simulink model "dab_openloop_variable_step"  (R2024b)
settings: Solver=ode1be  StartTime=0.0  StopTime=T_stop  FixedStep=TFIX  MaxStep=Tsolver  RelTol=1e-05
values from neighbouring files (symbols this model uses):
  Ci = 30e-6*s_f    (= 7.5e-05)    [init.m]
  Co = 44e-6*s_f    (= 0.00011)    [init.m]
  D1_OL = 0.985714    [init.m]
  D2_OL = 1    [init.m]
  D3_OL = 0.045188    [init.m]
  ESR_Ci = 2e-3    (= 0.002)    [init.m]
  ESR_Co = 2e-3    (= 0.002)    [init.m]
  f_sw = 20e3    (= 20000)    [init.m]
  Li = 10e-6*s_f    (= 2.5e-05)    [init.m]
  Lo = 10e-6*s_f    (= 2.5e-05)    [init.m]
  Ri = 100e-3    (= 0.1)    [init.m]
  Ro = 100e-3    (= 0.1)    [init.m]
  tdead = 200e-9    (= 2e-07)    [init.m]
  TR_fn = f_sw    (= 20000)    [init.m]
  TR_Lm = 1    [init.m]
  TR_Pn = 30e3    (= 30000)    [init.m]
  TR_Rm = 1e6    (= 1000000)    [init.m]
  Vi = 800    [init.m]
  Vo = V_BAT    (= 450)    [init.m]
libraries: spsMosfetLib x8, spsSeriesRLCBranchLib x4, spsControlledVoltageSourceLib x2, spsCurrentMeasurementLib x2, spsGroundLib x2, spsVoltageMeasurementLib x2, spsLinearTransformerLib x1, sps_lib x1
settings Model: Creator=amina  LastModifiedBy=amina
settings SolverCC: MaxConsecutiveMinStep=100
settings DataIOCC: SaveOutput=off  SignalLogging=off  DSMLogging=off  SaveTime=off  ReturnWorkspaceOutputsName=out_analytic

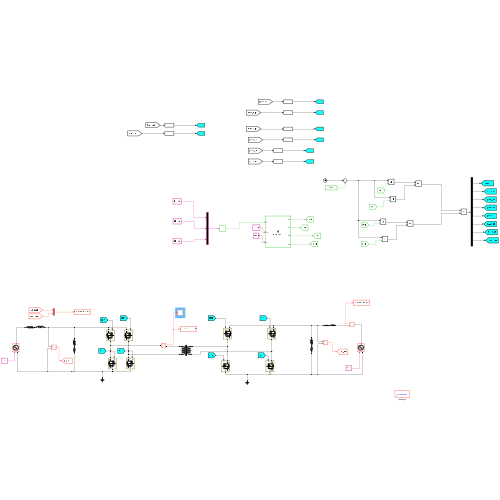
[thumbnail: Simulink's stored preview of the top-level diagram]
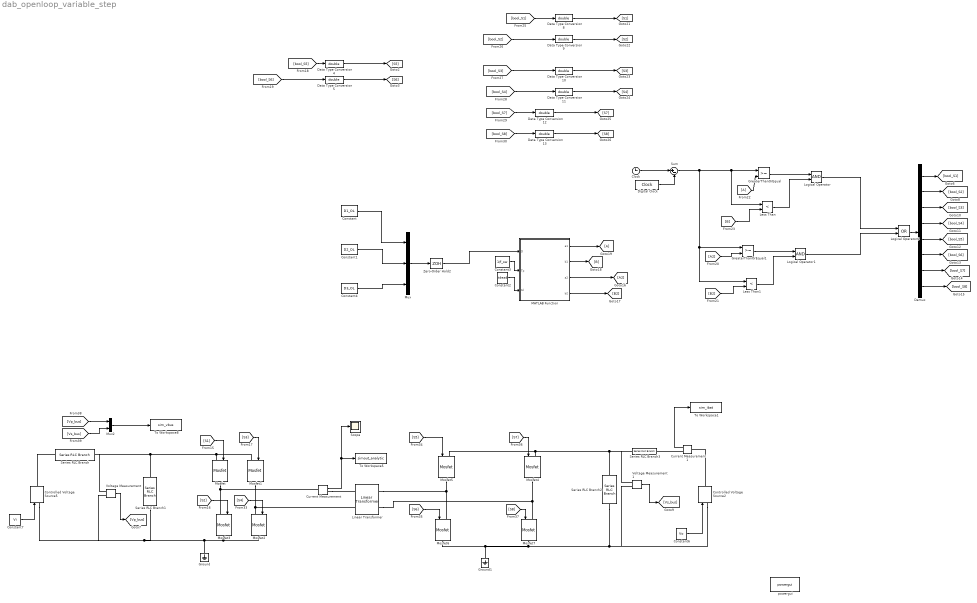
== system dab_openloop_variable_step ==
  Clock : Clock
  Constant : Constant  Value=D1_OL
  Constant1 : Constant  Value=D2_OL
  Constant2 : Constant  Value=tdead
  Constant3 : Constant  Value=1/f_sw
  Constant4 : Constant  Value=D3_OL
  Constant6 : Constant  Value=Vo
  Constant7 : Constant  Value=Vi
  Controlled Voltage Source2 : spsControlledVoltageSourceLib/Controlled Voltage Source  Initialize=on  Source_Type=DC  Amplitude=Vo  Phase=0  Frequency=0  Measurements=None
  Controlled Voltage Source5 : spsControlledVoltageSourceLib/Controlled Voltage Source  Initialize=on  Source_Type=DC  Amplitude=Vi  Phase=0  Frequency=0  Measurements=None
  Current Measurement : spsCurrentMeasurementLib/Current Measurement  PhasorSimulation=off  OutputType=Complex  PSBequivalent=0
  Current Measurement1 : spsCurrentMeasurementLib/Current Measurement  PhasorSimulation=off  OutputType=Complex  PSBequivalent=0
  Data Type Conversion{4..5,8..13} (8 alike) : DataTypeConversion  OutDataTypeStr=double  SaturateOnIntegerOverflow=off  RndMeth=Floor
  Demux : Demux  Outputs=8
  Digital Clock : DigitalClock  SampleTime=1/f_sw
  From22 : From
  Goto19 : Goto
  GreaterThanOrEqual : RelationalOperator  OutDataTypeStr=boolean  RndMeth=Simplest  InputSameDT=off
  GreaterThanOrEqual1 : RelationalOperator  OutDataTypeStr=boolean  RndMeth=Simplest  InputSameDT=off
  Ground : spsGroundLib/Ground  LConnTagsString=a
  Ground1 : spsGroundLib/Ground  LConnTagsString=a
  Less Than : RelationalOperator  Operator=<  OutDataTypeStr=boolean  RndMeth=Simplest  InputSameDT=off
  Less Than1 : RelationalOperator  Operator=<  OutDataTypeStr=boolean  RndMeth=Simplest  InputSameDT=off
  Linear Transformer : spsLinearTransformerLib/Linear Transformer  UNITS=SI  NominalPower=[TR_Pn TR_fn]  winding1=TR_W1  winding2=TR_W2  ThreeWindings=off  winding3=[3.15e+05 0.7938 0.084225]  RmLm=[TR_Rm TR_Lm]  Measurements=None  DataType=on
  Logical Operator : Logic  AllPortsSameDT=off  OutDataTypeStr=boolean
  Logical Operator1 : Logic  AllPortsSameDT=off  OutDataTypeStr=boolean
  Logical Operator6 : Logic  Operator=OR  AllPortsSameDT=off  OutDataTypeStr=boolean
  MATLAB Function : MATLAB Function  TreatAsAtomicUnit=on
  Mosfet{,1..7} (8 alike) : spsMosfetLib/Mosfet  Ron=Ron  Lon=0  Rd=Rd_diode  Vfd=Vf_diode  IC=0  Rs=Rs_snub  Cs=Cs_snub  Measurements=off
  Mux : Mux  Inputs=3
  Mux2 : Mux  Inputs=2
  Scope : Scope
  Series RLC Branch : spsSeriesRLCBranchLib/Series RLC Branch  LConnTagsString=__new0  RConnTagsString=__new0  BranchType=RL  Resistance=Ri  Inductance=Li  SetiL0=on  InitialCurrent=IL0_i  Capacitance=1e-6  Setx0=off  InitialVoltage=0  Measurements=None
  Series RLC Branch1 : spsSeriesRLCBranchLib/Series RLC Branch  LConnTagsString=__new0  RConnTagsString=__new0  BranchType=RC  Resistance=ESR_Ci  Inductance=1e-3  SetiL0=off  InitialCurrent=0  Capacitance=Ci  Setx0=on  InitialVoltage=V_cap_init  Measurements=None
  Series RLC Branch2 : spsSeriesRLCBranchLib/Series RLC Branch  LConnTagsString=__new0  RConnTagsString=__new0  BranchType=RC  Resistance=ESR_Co  Inductance=1e-3  SetiL0=off  InitialCurrent=0  Capacitance=Co  Setx0=on  InitialVoltage=V_out_init  Measurements=None
  Series RLC Branch3 : spsSeriesRLCBranchLib/Series RLC Branch  LConnTagsString=__new0  RConnTagsString=__new0  BranchType=RL  Resistance=Ro  Inductance=Lo  SetiL0=on  InitialCurrent=IL0_o  Capacitance=1e-6  Setx0=off  InitialVoltage=0  Measurements=None
  Sum : Sum  Inputs=|+-
  To Workspace1 : ToWorkspace  VariableName=sim_ibat  SaveFormat=Timeseries  SampleTime=-1
  To Workspace5 : ToWorkspace  VariableName=simout_analytic  SaveFormat=Timeseries  SampleTime=-1
  To Workspace8 : ToWorkspace  VariableName=sim_vbus  SaveFormat=Timeseries  SampleTime=-1
  Voltage Measurement : spsVoltageMeasurementLib/Voltage Measurement  PhasorSimulation=off  OutputType=Complex  PSBequivalent=0
  Voltage Measurement1 : spsVoltageMeasurementLib/Voltage Measurement  PhasorSimulation=off  OutputType=Complex  PSBequivalent=0
  Zero-Order Hold2 : ZeroOrderHold  SampleTime=1/f_sw
  powergui : sps_lib/powergui  Priority=1  SimulationMode=Continuous  SampleTime=50e-6  frequency=60  Iterations=50  frequencyindice=0  Pbase=100e6  ErrMax=1e-4  UnitsV=kV  UnitsW=MW  buscounter=0  FunctionMessages=off  echomessages=off  EnableUseOfTLC=off  CurrentSourceSwitches=off  DisableSnubberDevices=off  DisableRonSwitches=off  DisableVfSwitches=off  DisplayEquations=off  AutomaticDiscreteSolvers=off  SolverType=Tustin/Backward Euler (TBE)  Interpol=off  ExternalGateDelay=off  methode=off  Ts=100  x0status=blocks  SPID=on  SwTol=0  HookPort=off  NonlinearTolerance=1e-4  nMaxIteration=100  ContinueOnMaxIteration=off  RestoreLinks=warning  ResistiveCurrentMeasurement=off  Frange=[0:2:500]  Ylog=off  Xlog=on  ShowGrid=off  save=off  variable=ZData  structure=0  ZoomFFT=off  StartTime=0.0  cycles=1  DisplayStyle=1  fundamental=60  FreqAxis=off  MaxFrequency=1000  frequencyindicesteady=1  RmsSteady=1  display=off
  wires:
  Constant/1 -> Mux/1
  Constant1/1 -> Mux/2
  Constant4/1 -> Mux/3
  Mux/1 -> Zero-Order Hold2/1
  Constant3/1 -> MATLAB Function/2(Tp)
  Zero-Order Hold2/1 -> MATLAB Function/1(D)
  Constant2/1 -> MATLAB Function/3(td)
  Clock/1 -> Sum/1
  Digital Clock/1 -> Sum/2
  Sum/1 -> Less Than1/1, GreaterThanOrEqual1/1, GreaterThanOrEqual/1, Less Than/1
  GreaterThanOrEqual/1 -> Logical Operator/1
  Less Than/1 -> Logical Operator/2
  [bool_S6] -> Data Type Conversion5/1
  Data Type Conversion5/1 -> [S6]
  Data Type Conversion4/1 -> [S5]
  [bool_S5] -> Data Type Conversion4/1
  MATLAB Function/1(a1) -> Goto19/1
  MATLAB Function/2(b1) -> [B]
  From22/1 -> GreaterThanOrEqual/2
  [B] -> Less Than/2
  Demux/5 -> [bool_S5]
  Demux/1 -> [bool_S1]
  Demux/8 -> [bool_S8]
  Demux/7 -> [bool_S7]
  Demux/6 -> [bool_S6]
  Demux/4 -> [bool_S4]
  Demux/2 -> [bool_S2]
  Demux/3 -> [bool_S3]
  Logical Operator6/1 -> Demux/1
  MATLAB Function/3(a2) -> [A2]
  MATLAB Function/4(b2) -> [B2]
  GreaterThanOrEqual1/1 -> Logical Operator1/1
  [B2] -> Less Than1/2
  [A2] -> GreaterThanOrEqual1/2
  Less Than1/1 -> Logical Operator1/2
  Logical Operator/1 -> Logical Operator6/1
  Logical Operator1/1 -> Logical Operator6/2
  Data Type Conversion11/1 -> [S4]
  Data Type Conversion13/1 -> [S8]
  [bool_S1] -> Data Type Conversion8/1
  [bool_S3] -> Data Type Conversion10/1
  [bool_S2] -> Data Type Conversion9/1
  [bool_S7] -> Data Type Conversion12/1
  Data Type Conversion9/1 -> [S2]
  Data Type Conversion10/1 -> [S3]
  Data Type Conversion8/1 -> [S1]
  [bool_S8] -> Data Type Conversion13/1
  Data Type Conversion12/1 -> [S7]
  [bool_S4] -> Data Type Conversion11/1
  Constant6/1 -> Controlled Voltage Source2/1
  Constant7/1 -> Controlled Voltage Source5/1
  Current Measurement/1 -> Scope/1, To Workspace5/1
  [S1] -> Mosfet/1
  [S2] -> Mosfet3/1
  [S3] -> Mosfet1/1
  [S4] -> Mosfet2/1
  [S6] -> Mosfet6/1
  [S5] -> Mosfet5/1
  [S7] -> Mosfet4/1
  [S8] -> Mosfet7/1
  Voltage Measurement/1 -> [Vp_bus]
  Voltage Measurement1/1 -> [Vs_bus]
  [Vs_bus] -> Mux2/2
  Mux2/1 -> To Workspace8/1
  [Vp_bus] -> Mux2/1
  Current Measurement1/1 -> To Workspace1/1
  connections:
  Mosfet/RConn1 -- Current Measurement/LConn1 -- Mosfet3/LConn1
  Mosfet/LConn1 -- Mosfet1/LConn1 -- Voltage Measurement/LConn1 -- Series RLC Branch/RConn1 -- Series RLC Branch1/LConn1
  Mosfet2/RConn1 -- Voltage Measurement/LConn2 -- Controlled Voltage Source5/LConn1 -- Series RLC Branch1/RConn1 -- Ground/LConn1 -- Mosfet3/RConn1
  Mosfet1/RConn1 -- Linear Transformer/LConn2 -- Mosfet2/LConn1
  Mosfet4/LConn1 -- Voltage Measurement1/LConn1 -- Series RLC Branch3/LConn1 -- Series RLC Branch2/LConn1 -- Mosfet5/LConn1
  Mosfet6/RConn1 -- Voltage Measurement1/LConn2 -- Controlled Voltage Source2/LConn1 -- Series RLC Branch2/RConn1 -- Mosfet7/RConn1 -- Ground1/LConn1
  Mosfet4/RConn1 -- Mosfet7/LConn1 -- Linear Transformer/RConn2
  Mosfet5/RConn1 -- Linear Transformer/RConn1 -- Mosfet6/LConn1
  Current Measurement/RConn1 -- Linear Transformer/LConn1
  Current Measurement1/RConn1 -- Series RLC Branch3/RConn1
  Controlled Voltage Source2/RConn1 -- Current Measurement1/LConn1
  Controlled Voltage Source5/RConn1 -- Series RLC Branch/LConn1

== matlab function dab_openloop_variable_step/MATLAB Function ==
  settings: updateMethod=DISCRETE  sampleTime=1/f_sw
  data: D input; a1 output size=[8 1]; Tp input; td input; b1 output size=[8 1]; a2 output size=[8 1]; b2 output size=[8 1]
function [a1, b1, a2, b2] = gate_block(D, Tp, td)
    persistent s0 p
    if isempty(s0)
        cu = [0; D(1); D(3); D(3) + D(2)];
        u  = mod(cu*Tp/2, Tp);   d = mod((cu + 1)*Tp/2, Tp);
        s0 = u > d;   p = max(u, d) - Tp;
    end
    [a1, b1, a2, b2, s0, p] = gate_core(D, Tp, td, s0, p);
end
